simulink model "VehiclePlant"  (R2026b)
settings: Solver=ode4  StopTime=60  FixedStep=0.01
undefined symbols (not defined in the file): DragCoeff, Mass
settings Model: DataDictionary=CruiseControlData.sldd  Creator=kingc  LastModifiedBy=kingc
settings ModelReferenceCC: ModelReferenceMinAlgLoopOccurrences=on

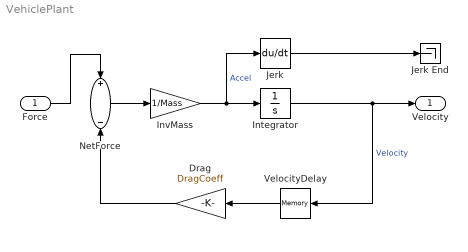
== system VehiclePlant ==
  Force : Inport
  Drag : Gain  Gain=DragCoeff
  Integrator : Integrator
  InvMass : Gain  Gain=1/Mass
  Jerk : Derivative
  Jerk End : Terminator
  NetForce : Sum  Inputs=+|-
  VelocityDelay : Memory
  Velocity : Outport
  wires:
  Force/1 -> NetForce/1
  NetForce/1 -> InvMass/1
  InvMass/1 -> Jerk/1, Integrator/1  "Accel"
  Integrator/1 -> VelocityDelay/1, Velocity/1  "Velocity"
  Jerk/1 -> Jerk End/1
  VelocityDelay/1 -> Drag/1
  Drag/1 -> NetForce/2
